simulink library "Prop_gryo"  (R2025b)
settings: Solver=VariableStepAuto  StartTime=0.0  StopTime=10.0  RelTol=1e-3
undefined symbols (not defined in the file): cfd2d_ja, cfd2d_jl, cfd2d_kQ, cfd2d_kT, cfd2d_P1_CEF_X, cfd2d_P1_CEF_Y, cfd2d_P1_CEF_Z, cfd2d_P1_CEM_X, cfd2d_P1_CEM_Y, cfd2d_P1_CEM_Z, cfd2d_P5_CEF_X, cfd2d_P5_CEF_Y, cfd2d_P5_CEF_Z, cfd2d_P5_CEM_X, cfd2d_P5_CEM_Y, cfd2d_P5_CEM_Z, cfd3d_ja, cfd3d_jl, cfd3d_kQ, cfd3d_kT, cfd3d_P2_CEF_X, cfd3d_P2_CEF_Y, cfd3d_P2_CEF_Z, cfd3d_P2_CEM_X, cfd3d_P2_CEM_Y, cfd3d_P2_CEM_Z, cfd3d_P6_CEF_X, cfd3d_P6_CEF_Y, cfd3d_P6_CEF_Z, cfd3d_P6_CEM_X, cfd3d_P6_CEM_Y, cfd3d_P6_CEM_Z, cfd3d_pitch, magnitude
libraries: matrix_library x16
(part 2 of 2)

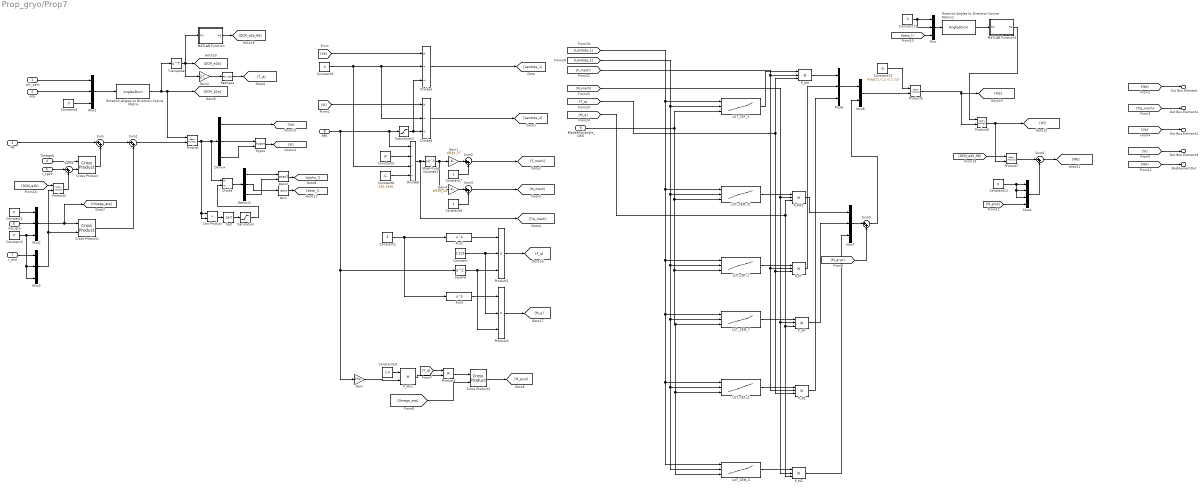
== system Prop_gryo/Prop7 ==
  phi_cant : Inport
  eta : Inport  Port=2
  Vb : Inport  Port=3
  Omegab : Inport  Port=4
  r_cg2k : Inport  Port=5
  dot_eta : Inport  Port=6
  r_arm : Inport  Port=7
  RPS : Inport  Port=8
  BladePitchAngle_DEG : Inport  Port=9
  Asin : Trigonometry  Operator=asin
  Atan2 : Trigonometry  Operator=atan2
  Constant : Constant  Value=1.225
  Constant1 : Constant  Value=3
  Constant10 : Constant  Value=1.0
  Constant{2..4,11..12} (5 alike) : Constant  Value=0
  Constant13 : Constant  Value=diag([1,-1,1,-1,1,-1])
  Constant5 : Constant  Value=pi
  Constant6 : Constant  Value=340.2940
  Constant7 : Constant
  Constant8 : Constant
  Constant9 : Constant  Value=3
  Cross Product : matrix_library/Cross Product
  Cross Product1 : matrix_library/Cross Product
  Cross Product2 : matrix_library/Cross Product
  Demux : Demux  Outputs=3
  Demux1 : Demux  Outputs=3
  Divide : Product  Inputs=*/
  Divide4 : Product  Inputs=*//
  Divide5 : Product  Inputs=*//
  Divide6 : Product  Inputs=***/
  Dot Product : DotProduct  OutDataTypeStr=Inherit: Inherit via internal rule
  Fcn2 : Fcn  Expr=u^4
  Fcn3 : Fcn  Expr=u^5
  Gain : Gain  Gain=2*pi
  Gain1 : Gain  Gain=cfd3d_kT
  Gain2 : Gain  Gain=[1 0 0]  Multiplication=Matrix(K*u)
  Gain4 : Gain  Gain=cfd3d_kQ
  Hypot : Math  Operator=hypot
  LUT_CEF_X : Lookup_n-D  NumberOfTableDimensions=3  BreakpointsForDimension1=cfd3d_ja  BreakpointsForDimension2=cfd3d_jl  BreakpointsForDimension3=cfd3d_pitch  Table=cfd3d_P6_CEF_X  UseLastTableValue=on  InternalRulePriority=Speed  RndMeth=Simplest
      settings: InputPortMap=u0,u1,u2
  LUT_CEF_Y : Lookup_n-D  NumberOfTableDimensions=3  BreakpointsForDimension1=cfd3d_ja  BreakpointsForDimension2=cfd3d_jl  BreakpointsForDimension3=cfd3d_pitch  Table=cfd3d_P6_CEF_Y  UseLastTableValue=on  InternalRulePriority=Speed  RndMeth=Simplest
      settings: InputPortMap=u0,u1,u2
  LUT_CEF_Z : Lookup_n-D  NumberOfTableDimensions=3  BreakpointsForDimension1=cfd3d_ja  BreakpointsForDimension2=cfd3d_jl  BreakpointsForDimension3=cfd3d_pitch  Table=cfd3d_P6_CEF_Z  UseLastTableValue=on  InternalRulePriority=Speed  RndMeth=Simplest
      settings: InputPortMap=u0,u1,u2
  LUT_CEM_X1 : Lookup_n-D  NumberOfTableDimensions=3  BreakpointsForDimension1=cfd3d_ja  BreakpointsForDimension2=cfd3d_jl  BreakpointsForDimension3=cfd3d_pitch  Table=cfd3d_P6_CEM_X  UseLastTableValue=on  InternalRulePriority=Speed  RndMeth=Simplest
      settings: InputPortMap=u0,u1,u2
  LUT_CEM_Y : Lookup_n-D  NumberOfTableDimensions=3  BreakpointsForDimension1=cfd3d_ja  BreakpointsForDimension2=cfd3d_jl  BreakpointsForDimension3=cfd3d_pitch  Table=cfd3d_P6_CEM_Y  UseLastTableValue=on  InternalRulePriority=Speed  RndMeth=Simplest
      settings: InputPortMap=u0,u1,u2
  LUT_CEM_Z : Lookup_n-D  NumberOfTableDimensions=3  BreakpointsForDimension1=cfd3d_ja  BreakpointsForDimension2=cfd3d_jl  BreakpointsForDimension3=cfd3d_pitch  Table=cfd3d_P6_CEM_Z  UseLastTableValue=on  InternalRulePriority=Speed  RndMeth=Simplest
      settings: InputPortMap=u0,u1,u2
  MATLAB Function : MATLAB Function  TreatAsAtomicUnit=on
  MATLAB Function1 : MATLAB Function  TreatAsAtomicUnit=on
  Magnitude Squared1 : Math  Operator=magnitude^2
  Mux{,1..3,6..7} (6 alike) : Mux  Inputs=3
  Mux4 : Mux
  Mux8 : Mux  Inputs=2
  P_FY : Product  Inputs=***
  P_FZ : Product  Inputs=***
  P_MX : Product  Inputs=***
  P_MX1 : Product  Inputs=***
  P_MY : Product  Inputs=***
  P_MY1 : Product  Inputs=**
  P_MZ : Product  Inputs=***
  Product{,2,5..7} (5 alike) : Product  Multiplication=Matrix(*)
  Product1 : Product  Inputs=3
  Product3 : Product  Inputs=3
  Product4 : Product
  Reshape : Reshape
  Rotation Angles to Direction Cosine Matrix : Angle2Dcm  rotationOrder=XYZ
      settings: AttributesFormatString=Rotation Order: %<rotationOrder>
  Rotation Angles to Direction Cosine Matrix1 : Angle2Dcm  rotationOrder=XYZ
      settings: AttributesFormatString=Rotation Order: %<rotationOrder>
  Saturation : Saturate  UpperLimit=inf  LowerLimit=1e-4
  Saturation2 : Saturate  UpperLimit=10000  LowerLimit=0.0001
  Sqrt : Sqrt
  Square : Math  Operator=square
  Sum{,1..6} (7 alike) : Sum  Inputs=|++
  Transpose : Math  Operator=transpose
  Out Bus Element : Outport  PortName=Prop  Element=Wp
  Out Bus Element1 : Outport  PortName=Prop  Element=Tip_mach
  Out Bus Element2 : Outport  PortName=Prop  Element=Va
  Out Bus Element3 : Outport  PortName=Prop  Element=Vl
  BusElementOut : Outport  PortName=Prop  Element=Wb
  wires:
  Constant4/1 -> Mux1/3
  Demux/3 -> Hypot/2
  Hypot/1 -> [Vl]
  LUT_CEF_Y/1 -> P_FY/1
  Mux7/1 -> Sum5/1
  LUT_CEF_X/1 -> P_MX/1
  Mux6/1 -> Mux8/1
  P_MX/1 -> Mux6/1
  LUT_CEM_X1/1 -> P_MX1/1
  LUT_CEF_Z/1 -> P_FZ/1
  Sum4/1 -> Cross Product/2
  Constant2/1 -> Mux2/1
  Omegab/1 -> Cross Product/1
  [F_q] -> P_MX/3, P_FY/3, P_FZ/3
  Constant6/1 -> Divide6/4
  [Lambda_1] -> LUT_CEM_X1/1, LUT_CEF_Y/1, LUT_CEM_Y/1, LUT_CEF_Z/1, LUT_CEM_Z/1, LUT_CEF_X/1
  Vb/1 -> Sum/1
  Mux1/1 -> Rotation Angles to Direction Cosine Matrix/1
  Gain4/1 -> Sum3/1
  Square/1 -> Product1/3, Product3/3
  BladePitchAngle_DEG/1 -> LUT_CEF_X/3, LUT_CEM_X1/3, LUT_CEF_Y/3, LUT_CEM_Y/3, LUT_CEF_Z/3, LUT_CEM_Z/3
  Divide6/1 -> Magnitude Squared1/1, [Tip_mach]
  LUT_CEM_Z/1 -> P_MZ/1
  Product3/1 -> [M_q]
  RPS/1 -> Saturation2/1, Divide6/1, Gain/1, Square/1
  Divide4/1 -> [Lambda_2]
  Fcn2/1 -> Product1/1
  P_MY/1 -> Mux7/2
  Product2/1 -> Sum4/2
  [Va] -> Divide5/1
  r_cg2k/1 -> Sum4/1
  dot_eta/1 -> Mux2/2
  LUT_CEM_Y/1 -> P_MY/1
  phi_cant/1 -> Mux1/1
  Fcn3/1 -> Product3/1
  [F_mach] -> P_MX/2, P_FY/2, P_FZ/2
  Constant9/1 -> Divide5/2, Divide4/2, Divide6/3
  Demux/1 -> [Va]
  Constant7/1 -> Sum2/2
  Sum2/1 -> [F_mach]
  [M_q] -> P_MX1/3, P_MY/3, P_MZ/3
  Demux/2 -> Hypot/1
  [Vl] -> Divide4/1
  [M_mach] -> P_MX1/2, P_MY/2, P_MZ/2
  Product1/1 -> [F_q]
  Sum/1 -> Sum1/1
  Cross Product1/1 -> Sum1/2
  Sum3/1 -> [M_mach]
  [Lambda_2] -> LUT_CEF_X/2, LUT_CEM_X1/2, LUT_CEF_Y/2, LUT_CEM_Y/2, LUT_CEF_Z/2, LUT_CEM_Z/2
  Constant5/1 -> Divide6/2
  Divide5/1 -> [Lambda_1]
  Mux3/1 -> Product2/2, Cross Product1/2
  P_FZ/1 -> Mux6/3
  [DCM_e2b] -> Product2/1
  Rotation Angles to Direction Cosine Matrix/1 -> [DCM_b2e], Product/1, Transpose/1
  Sum1/1 -> Product/2
  Cross Product/1 -> Sum/2
  Magnitude Squared1/1 -> Gain1/1, Gain4/1
  Gain1/1 -> Sum2/1
  r_arm/1 -> Mux3/1
  Constant8/1 -> Sum3/2
  Saturation2/1 -> Divide4/3, Divide5/3
  Constant/1 -> Product1/2, Product3/2
  Constant3/1 -> Mux2/3, Mux3/2, Mux3/3
  eta/1 -> Mux1/2
  Constant1/1 -> Fcn2/1, Fcn3/1
  Sum5/1 -> Mux8/2
  [M_gryo] -> Sum5/2
  P_MY1/1 -> Product4/2
  Cross Product2/1 -> [M_gryo]
  [T_A] -> Product4/1
  Constant10/1 -> P_MY1/1
  Product4/1 -> Cross Product2/1
  Gain/1 -> P_MY1/2
  Gain2/1 -> Reshape/1
  [Omega_eta] -> Cross Product2/2
  Mux2/1 -> [Omega_eta], Cross Product1/1
  Product5/1 -> Product6/2, [Wp]
  Constant11/1 -> Mux/2, Mux/1
  [DCM_e2b_R6] -> Product7/1
  [Wb] -> BusElementOut/1
  Mux/1 -> Rotation Angles to Direction Cosine Matrix1/1
  Product6/1 -> [Wl], Product7/2
  [Va] -> Out Bus Element2/1
  Sum6/1 -> [Wb]
  [Wp] -> Out Bus Element/1
  Constant12/1 -> Mux4/3, Mux4/2, Mux4/1
  Product7/1 -> Sum6/1
  Mux4/1 -> Sum6/2
  [beta_l] -> Mux/3
  MATLAB Function1/1(R6) -> Product6/1
  Rotation Angles to Direction Cosine Matrix1/1 -> MATLAB Function1/1(R3)
  [Tip_mach] -> Out Bus Element1/1
  [M_gryo] -> Mux4/4
  [Vl] -> Out Bus Element3/1
  MATLAB Function/1(R6) -> [DCM_e2b_R6]
  Transpose/1 -> [DCM_e2b], Gain2/1, MATLAB Function/1(R3)
  Mux8/1 -> Product5/2
  Constant13/1 -> Product5/1
  Reshape/1 -> [T_A]
  Dot Product/1 -> Sqrt/1
  Sqrt/1 -> Saturation/1
  Demux1/2 -> Asin/1
  Atan2/1 -> [alpha_l]
  Product/1 -> Divide/1, Demux/1, Dot Product/1, Dot Product/2
  Asin/1 -> [beta_l]
  Demux1/1 -> Atan2/1
  Divide/1 -> Demux1/1
  Demux1/3 -> Atan2/2
  Saturation/1 -> Divide/2
  P_FY/1 -> Mux6/2
  P_MX1/1 -> Mux7/1
  P_MZ/1 -> Mux7/3

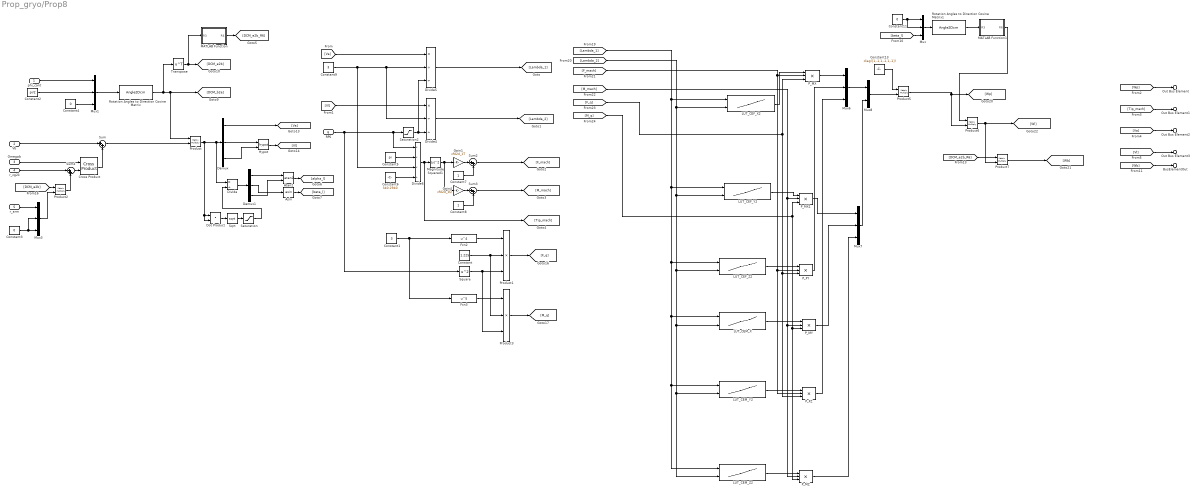
== system Prop_gryo/Prop8 ==
  phi_cant : Inport
  Vb : Inport  Port=2
  Omegab : Inport  Port=3
  r_cg2k : Inport  Port=4
  r_arm : Inport  Port=5
  RPS : Inport  Port=6
  Asin : Trigonometry  Operator=asin
  Atan2 : Trigonometry  Operator=atan2
  Constant : Constant  Value=1.225
  Constant1 : Constant  Value=3
  Constant11 : Constant  Value=0
  Constant13 : Constant  Value=diag([1,-1,1,-1,1,-1])
  Constant2 : Constant  Value=pi/2
  Constant3 : Constant  Value=0
  Constant4 : Constant  Value=0
  Constant5 : Constant  Value=pi
  Constant6 : Constant  Value=340.2940
  Constant7 : Constant
  Constant8 : Constant
  Constant9 : Constant  Value=3
  Cross Product : matrix_library/Cross Product
  Demux : Demux  Outputs=3
  Demux1 : Demux  Outputs=3
  Divide : Product  Inputs=*/
  Divide4 : Product  Inputs=*//
  Divide5 : Product  Inputs=*//
  Divide6 : Product  Inputs=***/
  Dot Product : DotProduct  OutDataTypeStr=Inherit: Inherit via internal rule
  Fcn2 : Fcn  Expr=u^4
  Fcn3 : Fcn  Expr=u^5
  Gain1 : Gain  Gain=cfd2d_kT
  Gain4 : Gain  Gain=cfd2d_kQ
  Hypot : Math  Operator=hypot
  LUT_CEF_X2 : Lookup_n-D  BreakpointsForDimension1=cfd2d_ja  BreakpointsForDimension2=cfd2d_jl  BreakpointsForDimension3=[5, 7]  Table=cfd2d_P5_CEF_X  UseLastTableValue=on  InternalRulePriority=Speed  RndMeth=Simplest
      settings: InputPortMap=u0,u1
  LUT_CEF_Y2 : Lookup_n-D  BreakpointsForDimension1=cfd2d_ja  BreakpointsForDimension2=cfd2d_jl  BreakpointsForDimension3=[5, 7]  Table=cfd2d_P5_CEM_X  UseLastTableValue=on  InternalRulePriority=Speed  RndMeth=Simplest
      settings: InputPortMap=u0,u1
  LUT_CEF_Z2 : Lookup_n-D  BreakpointsForDimension1=cfd2d_ja  BreakpointsForDimension2=cfd2d_jl  BreakpointsForDimension3=[5, 7]  Table=cfd2d_P5_CEF_Y  UseLastTableValue=on  InternalRulePriority=Speed  RndMeth=Simplest
      settings: InputPortMap=u0,u1
  LUT_CEM_X : Lookup_n-D  BreakpointsForDimension1=cfd2d_ja  BreakpointsForDimension2=cfd2d_jl  BreakpointsForDimension3=[5, 7]  Table=cfd2d_P5_CEM_Y  UseLastTableValue=on  InternalRulePriority=Speed  RndMeth=Simplest
      settings: InputPortMap=u0,u1
  LUT_CEM_Y2 : Lookup_n-D  BreakpointsForDimension1=cfd2d_ja  BreakpointsForDimension2=cfd2d_jl  BreakpointsForDimension3=[5, 7]  Table=cfd2d_P5_CEF_Z  UseLastTableValue=on  InternalRulePriority=Speed  RndMeth=Simplest
      settings: InputPortMap=u0,u1
  LUT_CEM_Z2 : Lookup_n-D  BreakpointsForDimension1=cfd2d_ja  BreakpointsForDimension2=cfd2d_jl  BreakpointsForDimension3=[5, 7]  Table=cfd2d_P5_CEM_Z  UseLastTableValue=on  InternalRulePriority=Speed  RndMeth=Simplest
      settings: InputPortMap=u0,u1
  MATLAB Function : MATLAB Function  TreatAsAtomicUnit=on
  MATLAB Function1 : MATLAB Function  TreatAsAtomicUnit=on
  Magnitude Squared1 : Math  Operator=magnitude^2
  Mux{,1,3,6..7} (5 alike) : Mux  Inputs=3
  Mux8 : Mux  Inputs=2
  P_FY : Product  Inputs=***
  P_FZ : Product  Inputs=***
  P_MX : Product  Inputs=***
  P_MX1 : Product  Inputs=***
  P_MY : Product  Inputs=***
  P_MZ : Product  Inputs=***
  Product{,2,5..7} (5 alike) : Product  Multiplication=Matrix(*)
  Product1 : Product  Inputs=3
  Product3 : Product  Inputs=3
  Rotation Angles to Direction Cosine Matrix : Angle2Dcm  rotationOrder=XYZ
      settings: AttributesFormatString=Rotation Order: %<rotationOrder>
  Rotation Angles to Direction Cosine Matrix1 : Angle2Dcm  rotationOrder=XYZ
      settings: AttributesFormatString=Rotation Order: %<rotationOrder>
  Saturation : Saturate  UpperLimit=inf  LowerLimit=1e-4
  Saturation2 : Saturate  UpperLimit=10000  LowerLimit=0.0001
  Sqrt : Sqrt
  Square : Math  Operator=square
  Sum{,2..4} (4 alike) : Sum  Inputs=|++
  Transpose : Math  Operator=transpose
  Out Bus Element : Outport  PortName=Prop  Element=Wp
  Out Bus Element1 : Outport  PortName=Prop  Element=Tip_mach
  Out Bus Element2 : Outport  PortName=Prop  Element=Va
  Out Bus Element3 : Outport  PortName=Prop  Element=Vl
  BusElementOut : Outport  PortName=Prop  Element=Wb
  wires:
  Constant1/1 -> Fcn3/1, Fcn2/1
  Constant2/1 -> Mux1/2
  Constant3/1 -> Mux3/2, Mux3/3
  Constant/1 -> Product3/2, Product1/2
  Saturation2/1 -> Divide5/3, Divide4/3
  Constant8/1 -> Sum3/2
  r_arm/1 -> Mux3/1
  Gain1/1 -> Sum2/1
  Magnitude Squared1/1 -> Gain4/1, Gain1/1
  Cross Product/1 -> Sum/2
  Sum/1 -> Product/2
  [DCM_e2b] -> Product2/1
  P_FZ/1 -> Mux6/3
  Mux3/1 -> Product2/2
  Divide5/1 -> [Lambda_1]
  Constant5/1 -> Divide6/2
  [Lambda_2] -> LUT_CEF_X2/2, LUT_CEF_Y2/2, LUT_CEF_Z2/2, LUT_CEM_Z2/2, LUT_CEM_Y2/2, LUT_CEM_X/2
  Sum3/1 -> [M_mach]
  Product1/1 -> [F_q]
  [M_mach] -> P_MZ/2, P_MY/2, P_MX1/2
  [Vl] -> Divide4/1
  Demux/2 -> Hypot/1
  [M_q] -> P_MZ/3, P_MY/3, P_MX1/3
  Sum2/1 -> [F_mach]
  Constant7/1 -> Sum2/2
  Demux/1 -> [Va]
  Constant9/1 -> Divide6/3, Divide4/2, Divide5/2
  [F_mach] -> P_FZ/2, P_FY/2, P_MX/2
  Fcn3/1 -> Product3/1
  phi_cant/1 -> Mux1/1
  LUT_CEM_X/1 -> P_MY/1
  r_cg2k/1 -> Sum4/1
  [Va] -> Divide5/1
  Product2/1 -> Sum4/2
  P_MY/1 -> Mux7/2
  Fcn2/1 -> Product1/1
  Divide4/1 -> [Lambda_2]
  RPS/1 -> Square/1, Divide6/1, Saturation2/1
  Product3/1 -> [M_q]
  LUT_CEM_Z2/1 -> P_MZ/1
  Divide6/1 -> [Tip_mach], Magnitude Squared1/1
  Square/1 -> Product3/3, Product1/3
  Gain4/1 -> Sum3/1
  Mux1/1 -> Rotation Angles to Direction Cosine Matrix/1
  Vb/1 -> Sum/1
  [Lambda_1] -> LUT_CEF_X2/1, LUT_CEF_Y2/1, LUT_CEF_Z2/1, LUT_CEM_Z2/1, LUT_CEM_Y2/1, LUT_CEM_X/1
  Constant6/1 -> Divide6/4
  Transpose/1 -> MATLAB Function/1(R3), [DCM_e2b]
  [F_q] -> P_FZ/3, P_FY/3, P_MX/3
  Omegab/1 -> Cross Product/1
  Sum4/1 -> Cross Product/2
  LUT_CEM_Y2/1 -> P_FZ/1
  LUT_CEF_Y2/1 -> P_MX1/1
  P_MX/1 -> Mux6/1
  Mux6/1 -> Mux8/1
  LUT_CEF_X2/1 -> P_MX/1
  Mux7/1 -> Mux8/2
  LUT_CEF_Z2/1 -> P_FY/1
  Hypot/1 -> [Vl]
  Demux/3 -> Hypot/2
  Constant4/1 -> Mux1/3
  MATLAB Function/1(R6) -> [DCM_e2b_R6]
  Rotation Angles to Direction Cosine Matrix/1 -> Transpose/1, Product/1, [DCM_b2e]
  [Vl] -> Out Bus Element3/1
  Rotation Angles to Direction Cosine Matrix1/1 -> MATLAB Function1/1(R3)
  [Tip_mach] -> Out Bus Element1/1
  MATLAB Function1/1(R6) -> Product6/1
  [beta_l] -> Mux/3
  [Wp] -> Out Bus Element/1
  Product6/1 -> [Wl], Product7/2
  Constant11/1 -> Mux/2, Mux/1
  [Wb] -> BusElementOut/1
  [DCM_e2b_R6] -> Product7/1
  [Va] -> Out Bus Element2/1
  Mux/1 -> Rotation Angles to Direction Cosine Matrix1/1
  Product5/1 -> Product6/2, [Wp]
  Product7/1 -> [Wb]
  Mux8/1 -> Product5/2
  Constant13/1 -> Product5/1
  Dot Product/1 -> Sqrt/1
  Sqrt/1 -> Saturation/1
  Demux1/2 -> Asin/1
  Atan2/1 -> [alpha_l]
  Product/1 -> Dot Product/2, Dot Product/1, Divide/1, Demux/1
  Asin/1 -> [beta_l]
  Demux1/1 -> Atan2/1
  Divide/1 -> Demux1/1
  Demux1/3 -> Atan2/2
  Saturation/1 -> Divide/2
  P_FY/1 -> Mux6/2
  P_MX1/1 -> Mux7/1
  P_MZ/1 -> Mux7/3

== matlab function Prop_gryo/Prop4/MATLAB Function1 ==
  data: R3 input; R6 output
function R6 = fcn(R3)
    R6 = blkdiag(R3, R3);
end

== matlab function Prop_gryo/Prop8/MATLAB Function1 ==
  data: R3 input; R6 output
function R6 = fcn(R3)
    R6 = blkdiag(R3, R3);
end

== matlab function Prop_gryo/Prop2/MATLAB Function ==
  data: R3 input; R6 output
function R6 = fcn(R3)
    R6 = blkdiag(R3, R3);
end

== matlab function Prop_gryo/Prop3/MATLAB Function1 ==
  data: R3 input; R6 output
function R6 = fcn(R3)
    R6 = blkdiag(R3, R3);
end

== matlab function Prop_gryo/Prop3/MATLAB Function ==
  data: R3 input; R6 output
function R6 = fcn(R3)
    R6 = blkdiag(R3, R3);
end

== matlab function Prop_gryo/Prop6/MATLAB Function1 ==
  data: R3 input; R6 output
function R6 = fcn(R3)
    R6 = blkdiag(R3, R3);
end

== matlab function Prop_gryo/Prop6/MATLAB Function ==
  data: R3 input; R6 output
function R6 = fcn(R3)
    R6 = blkdiag(R3, R3);
end

== matlab function Prop_gryo/Prop7/MATLAB Function1 ==
  data: R3 input; R6 output
function R6 = fcn(R3)
    R6 = blkdiag(R3, R3);
end

== matlab function Prop_gryo/Prop7/MATLAB Function ==
  data: R3 input; R6 output
function R6 = fcn(R3)
    R6 = blkdiag(R3, R3);
end

== matlab function Prop_gryo/Prop1/MATLAB Function1 ==
  data: R3 input; R6 output
function R6 = fcn(R3)
    R6 = blkdiag(R3, R3);
end

== matlab function Prop_gryo/Prop2/MATLAB Function1 ==
  data: R3 input; R6 output
function R6 = fcn(R3)
    R6 = blkdiag(R3, R3);
end

== matlab function Prop_gryo/Prop1/MATLAB Function ==
  data: R3 input; R6 output
function R6 = fcn(R3)
    R6 = blkdiag(R3, R3);
end

== matlab function Prop_gryo/Prop5/MATLAB Function ==
  data: R3 input; R6 output
function R6 = fcn(R3)
    R6 = blkdiag(R3, R3);
end

== matlab function Prop_gryo/Prop4/MATLAB Function ==
  data: R3 input; R6 output
function R6 = fcn(R3)
    R6 = blkdiag(R3, R3);
end

== matlab function Prop_gryo/Prop8/MATLAB Function ==
  data: R3 input; R6 output
function R6 = fcn(R3)
    R6 = blkdiag(R3, R3);
end

== matlab function Prop_gryo/Prop5/MATLAB Function1 ==
  data: R3 input; R6 output
function R6 = fcn(R3)
    R6 = blkdiag(R3, R3);
end
